simulink model "Stage1_Pipeline"  (R2026a)
settings: Solver=VariableStepAuto
libraries: visionsources x1
settings Model: Creator=adity  LastModifiedBy=adity

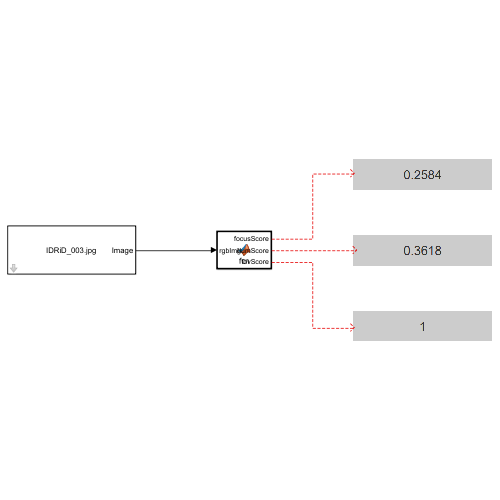
[thumbnail: Simulink's stored preview of the top-level diagram]
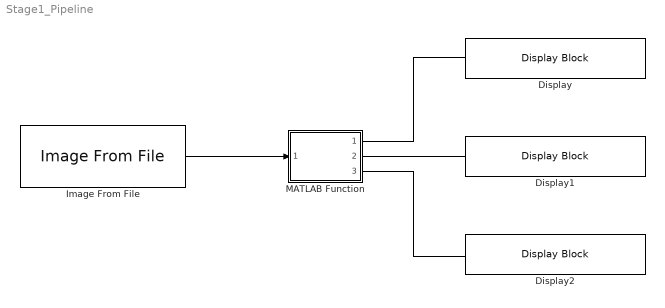
== system Stage1_Pipeline ==
  Display : DisplayBlock  LabelPosition=Hide  Transparency=1  GridColor=[0.502, 0.502, 0.502]
  Display1 : DisplayBlock  LabelPosition=Hide  Transparency=1  GridColor=[0.502, 0.502, 0.502]
  Display2 : DisplayBlock  LabelPosition=Hide  Transparency=1  GridColor=[0.502, 0.502, 0.502]
  Image From File : visionsources/Image From File  Tag=vipblks_nd  FileName=D:\IDRid dataset\Imagenes\Imagenes\IDRiD_003.jpg  Ts=inf  imagePorts=One multidimensional signal  OutPortLabels=R|G|B  ImageDataType=Inherit from input image  sdImageDataType=uint(8)  Signed=on  WordLength=16  FractionLengthMode=User-defined  FractionLength=15
  MATLAB Function : MATLAB Function  TreatAsAtomicUnit=on
  wires:
  Image From File/1 -> MATLAB Function/1(rgbImg)
  MATLAB Function/2(illumScore) -> ?
  MATLAB Function/1(focusScore) -> ?
  MATLAB Function/3(fovScore) -> ?

== matlab function Stage1_Pipeline/MATLAB Function ==
  data: rgbImg input; focusScore output; illumScore output; fovScore output
function [focusScore, illumScore, fovScore] = fcn(rgbImg)
%#codegen
grayImg = rgb2gray(rgbImg);
focusScore = computeFocusScore(grayImg);
illumScore = computeIlluminationScore(rgbImg);
fovScore = computeFOVScore(rgbImg);
end
